simulink model "Regenerative_Brakes_PMSM"  (R2024a)
settings: Solver=ode45  StartTime=0.0  StopTime=2.5  RelTol=1e-3  EnableMultiTasking=on
undefined symbols (not defined in the file): Ion, Lithium, sigbuilder_block
libraries: spsBatteryLib x1, AC7DriveInternalModels x1, spsPermanentMagnetSynchronousMachineLib x1, spsSeriesRLCBranchLib x1, spsThreePhaseFaultLib x1, spsUniversalBridgeLib x1, spspowerguiLib x1
settings Model: Creator=noname  LastModifiedBy=hirah
settings SolverCC: AlgebraicLoopSolver=TrustRegion
settings DataIOCC: LimitDataPoints=on  SaveFormat=Array  ReturnWorkspaceOutputs=off
settings OptimizationCC: LifeSpan=inf
settings DebuggingCC: UnderspecifiedInitializationDetection=Classic  MergeDetectMultiDrivingBlocksExec=none  SolverPrmCheckMsg=warning  UnconnectedInputMsg=warning  UnconnectedOutputMsg=warning  UnconnectedLineMsg=warning  StateNameClashWarn=warning  SFUnexpectedBacktrackingDiag=warning  SFNoUnconditionalDefaultTransitionDiag=warning  SFExecutionAtInitializationDiag=none  ArithmeticOperatorsInVariantConditions=warning
settings HardwareCC: ProdBitPerPointer=32  ProdBitPerSizeT=32  ProdBitPerPtrDiffT=32  ProdLargestAtomicFloat=None  ProdIntDivRoundTo=Undefined  ProdEndianess=Unspecified  ProdWordSize=32  ProdHWDeviceType=32-bit Generic
settings ModelReferenceCC: EnableRefExpFcnMdlSchedulingChecks=on  PropagateSignalLabelsOutOfModel=off
settings SFSimCC: SimUseLocalCustomCode=off  CustomCodeUndefinedFunction=UseInterfaceOnly
settings RTWCC: RTWUseLocalCustomCode=off  GPUComputeCapability=3.5  DLArmComputeVersion=19.05
settings CodeAppCC: StateflowObjectComments=on
settings GRTTargetCC: TargetLangStandard=C89/C90 (ANSI)
settings ConfigComp: CovMetricSettings=dw  CovSaveCumulativeToWorkspaceVar=on  CovSaveSingleToWorkspaceVar=on  CovExternalEMLEnable=off
settings SimscapeCC: SimscapeNormalizeSystem=off

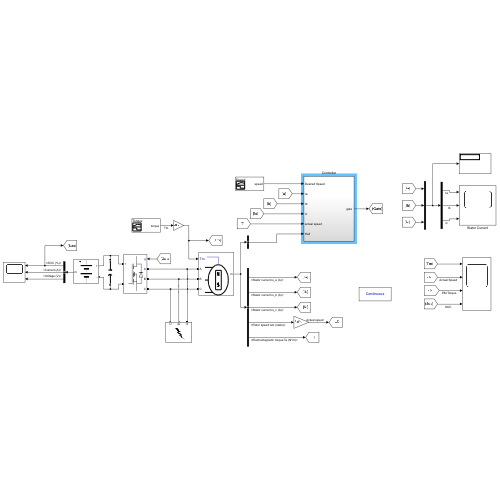
[thumbnail: Simulink's stored preview of the top-level diagram]
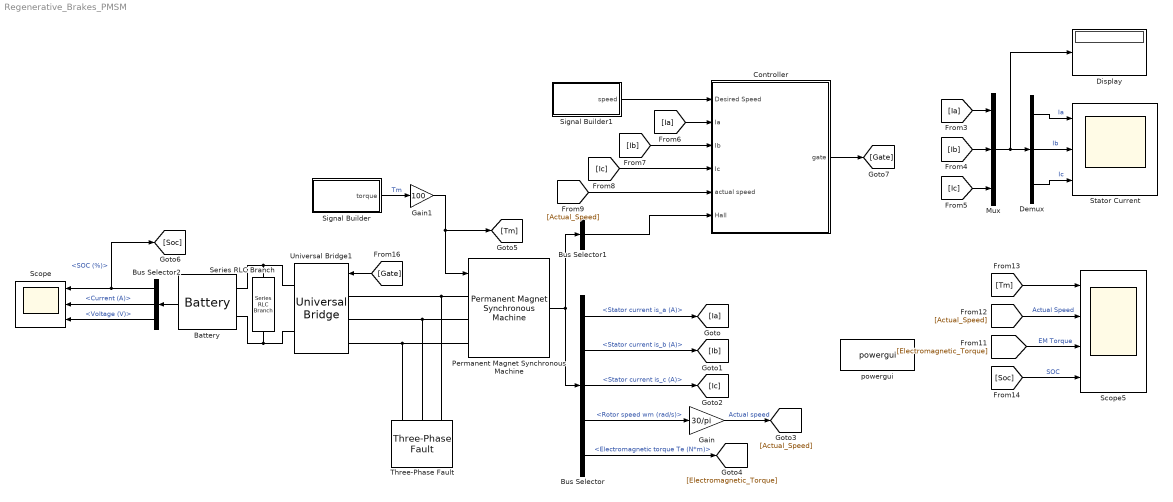
== system Regenerative_Brakes_PMSM ==
  Battery : spsBatteryLib/Battery  BatType=Lithium-Ion  ShowTempParam=off  ThermalPreset=no  ShowAgeParam=off  NomV=300  NomQ=100  SOC=80  Batt_Tr=30  PresetModel=off  MaxQ=84  MinV=215  FullV=330  Dis_rate=27.82608  R=0.006  Normal_OP=57.87524  expZone=[310 3.144344]  current=[1.5 3]  Units=Ampere-hour  Tci=20  NomT=20  T2=-30  MaxQ2=4.8  FullV2=7.1  Normal_OP2=5.655  expZone2="[6.58           1]"  Rca=0.6  ti=2000  Dp=0  Neq0=0  Tsim=1e6  Ta1=25  Qeol=5.4*0.9  Reol=0.013333*1.2  Char_age=[2.3478, 3]  Dis_age=[2.3478, 10]  N1=1500  N2=10500  N3=1000  N4=1400  Ta2=45  N5=950
  Bus Selector : BusSelector  OutputSignals=Stator current is_a (A),Stator current is_b (A),Stator current is_c (A),Rotor speed wm (rad/s),Electromagnetic torque Te (N*m)
  Bus Selector1 : BusSelector  OutputSignals=Hall effect signal h_a,Hall effect signal h_b,Hall effect signal h_c  OutputAsBus=on
  Bus Selector2 : BusSelector  OutputSignals=SOC (%),Current (A),Voltage (V)
  Controller : Subsystem
  Demux : Demux  Outputs=3
  Display : Display
  Gain : Gain  Gain=30/pi
  Gain1 : Gain  Gain=100
  Mux : Mux  Inputs=3
  Permanent Magnet Synchronous Machine : spsPermanentMagnetSynchronousMachineLib/Permanent Magnet Synchronous Machine  NbPhases=3  FluxDistribution=Sinusoidal  RotorType=Round  MechanicalLoad=Torque Tm  PresetModel="07:  20 Nm 300 Vdc 2200 RPM - 33.9 Nm"  ShowDetailedParameters=on  MeasurementBus=off  Resistance=0.129  Inductance=0.0144e-3  dqInductances=[8.5e-3,8.5e-3]  La=0.00153  MachineConstant=Flux linkage established by magnets (V.s)  Flux=0.1821  VoltageCst=132.1171  TorqueCst=1.0926  Flat=120  Mechanical=[0.003334 0.000425 4 0]  PolePairs=4  InitialConditions=[0,0, 0,0]  InitialConditions5ph=[0 0 0 0 0 0]  RefAngle=90 degrees behind phase A axis (modified Park)  IterativeDiscreteModel=Trapezoidal non iterative  TsBlock=-1  TsPowergui=0
  Scope : Scope  NumInputPorts=3
  Scope5 : Scope  NumInputPorts=4
  Series RLC Branch : spsSeriesRLCBranchLib/Series RLC Branch  LConnTagsString=__new0  RConnTagsString=__new0  BranchType=C  Resistance=1  Inductance=1e-3  SetiL0=off  InitialCurrent=0  Capacitance=75e-3  Setx0=off  InitialVoltage=0  Measurements=None
  Signal Builder : Subsystem  Tag=STV Subsys  LoadFcn=sigbuilder_block('load');  StartFcn=sigbuilder_block('start');  StopFcn=sigbuilder_block('stop');  ClipboardFcn=sigbuilder_block('clipboard');  mask(Sigbuilder block){tuvar=[0:10]}
      mask help: Simulink:masks:SigbuilderBlock_MD
      mask init:
      | if ~strcmp(get_param(bdroot(gcbh),'SimulationStatus'),'stopped') tuvar = sigbuilder_block('maskInit'); end
      settings: CopyFcn=sigbuilder_block('copy');  DeleteFcn=sigbuilder_block('delete');  ModelCloseFcn=sigbuilder_block('modelClose');  PreSaveFcn=sigbuilder_block('preSave');  PauseFcn=sigbuilder_block('pause');  ContinueFcn=sigbuilder_block('continue');  NameChangeFcn=sigbuilder_block('namechange');  OpenFcn=sigbuilder_block('open',[437.25 183.75 550.5 395.25 ]);  CloseFcn=sigbuilder_block('close');
      mask Display: plot(0, 0, 100, 100,[2, 2, 32, 32, 2], [68, 8, 8, 68, 68],[32, 2], [38, 38], [32, 19, 2],[53, 60, 44], [32, 17, 17, 2],[16, 16, 31, 31]);txt = getActiveGroup(gcbh);text(2, 100, txt,'verticalAlignment', 'top');
  Signal Builder1 : Subsystem  Tag=STV Subsys  LoadFcn=sigbuilder_block('load');  StartFcn=sigbuilder_block('start');  StopFcn=sigbuilder_block('stop');  ClipboardFcn=sigbuilder_block('clipboard');  mask(Sigbuilder block){tuvar=[0:10]}
      mask help: Simulink:masks:SigbuilderBlock_MD
      mask init:
      | if ~strcmp(get_param(bdroot(gcbh),'SimulationStatus'),'stopped') tuvar = sigbuilder_block('maskInit'); end
      settings: CopyFcn=sigbuilder_block('copy');  DeleteFcn=sigbuilder_block('delete');  ModelCloseFcn=sigbuilder_block('modelClose');  PreSaveFcn=sigbuilder_block('preSave');  PauseFcn=sigbuilder_block('pause');  ContinueFcn=sigbuilder_block('continue');  NameChangeFcn=sigbuilder_block('namechange');  OpenFcn=sigbuilder_block('open',[6.75 6.75 1138.5 568.5 ]);  CloseFcn=sigbuilder_block('close');
      mask Display: plot(0, 0, 100, 100,[2, 2, 32, 32, 2], [68, 8, 8, 68, 68],[32, 2], [38, 38], [32, 19, 2],[53, 60, 44], [32, 17, 17, 2],[16, 16, 31, 31]);txt = getActiveGroup(gcbh);text(2, 100, txt,'verticalAlignment', 'top');
  Stator Current : Scope  NumInputPorts=3
  Three-Phase Fault : spsThreePhaseFaultLib/Three-Phase Fault  InitialStates=0  FaultA=on  FaultB=on  FaultC=on  GroundFault=on  SwitchTimes="[1/60  5/60]"  External=off  SwitchStatus=NaN  FaultResistance=0.001  GroundResistance=0.01  SnubberResistance=1e6  SnubberCapacitance=inf  Measurements=None
  Universal Bridge1 : spsUniversalBridgeLib/Universal Bridge  Arms=3  SnubberResistance=1e5  SnubberCapacitance=inf  Device=MOSFET / Diodes  Ron=1e-3  Lon=0  ForwardVoltages="[  0  0  ]"  ForwardVoltage=0  GTOparameters=[ 10e-6 , 20e-6 ]  IGBTparameters=[ 1e-6 , 2e-6 ]  Measurements=None  Measurements_2=None  converterType=Rectifier
  powergui : spspowerguiLib/powergui  Priority=2  SimulationMode=Continuous  SampleTime=10e-6  frequency=60  Iterations=50  frequencyindice=0  Pbase=100e6  ErrMax=1e-4  UnitsV=kV  UnitsW=MW  buscounter=0  FunctionMessages=off  echomessages=off  EnableUseOfTLC=off  CurrentSourceSwitches=off  DisableSnubberDevices=off  DisableRonSwitches=off  DisableVfSwitches=off  DisplayEquations=off  AutomaticDiscreteSolvers=off  SolverType=Tustin  Interpol=off  ExternalGateDelay=off  methode=off  Ts=0  x0status=blocks  SPID=off  SwTol=0  HookPort=off  NonlinearTolerance=1e-4  nMaxIteration=100  ContinueOnMaxIteration=off  RestoreLinks=warning  ResistiveCurrentMeasurement=off  Frange=[0:2:500]  Ylog=off  Xlog=on  ShowGrid=off  save=off  variable=ZData  structure=N  ZoomFFT=off  StartTime=0.0  cycles=1  DisplayStyle=1  fundamental=60  FreqAxis=off  MaxFrequency=1000  frequencyindicesteady=1  RmsSteady=1  display=off
  wires:
  Permanent Magnet Synchronous Machine/1 -> Bus Selector/1, Bus Selector1/1
  Bus Selector/1 -> [Ia]  "<Stator current is_a (A)>"
  Bus Selector/2 -> [Ib]  "<Stator current is_b (A)>"
  Bus Selector/3 -> [Ic]  "<Stator current is_c (A)>"
  Bus Selector/4 -> Gain/1  "<Rotor speed wm (rad/s)>"
  Bus Selector1/1 -> Controller/6("Hall ")
  Gain/1 -> [Actual_Speed]  "Actual speed"
  Controller/1("gate ") -> [Gate]
  Battery/1 -> Bus Selector2/1
  Bus Selector2/1 -> Scope/1, [Soc]  "<SOC (%)>"
  Bus Selector2/2 -> Scope/2  "<Current (A)>"
  Bus Selector2/3 -> Scope/3  "<Voltage (V)>"
  Mux/1 -> Display/1, Demux/1
  Signal Builder/1(torque) -> Gain1/1  "Tm"
  Bus Selector/5 -> [Electromagnetic_Torque]  "<Electromagnetic torque Te (N*m)>"
  [Ia] -> Mux/1
  [Ib] -> Mux/2
  [Ic] -> Mux/3
  [Ia] -> Controller/2(Ia)
  [Ib] -> Controller/3(Ib)
  [Ic] -> Controller/4(Ic)
  [Actual_Speed] -> Controller/5(actual speed)
  [Actual_Speed] -> Scope5/2  "Actual Speed"
  [Tm] -> Scope5/1
  [Soc] -> Scope5/4  "SOC"
  [Gate] -> Universal Bridge1/1
  Signal Builder1/1(speed) -> Controller/1(Desired Speed)
  Demux/1 -> Stator Current/1  "Ia"
  Demux/2 -> Stator Current/2  "Ib"
  Demux/3 -> Stator Current/3  "Ic"
  [Electromagnetic_Torque] -> Scope5/3  "EM Torque"
  Gain1/1 -> Permanent Magnet Synchronous Machine/1, [Tm]
  connections:
  Universal Bridge1/LConn1 -- Three-Phase Fault/LConn1 -- Permanent Magnet Synchronous Machine/LConn1
  Permanent Magnet Synchronous Machine/LConn2 -- Universal Bridge1/LConn2 -- Three-Phase Fault/LConn2
  Universal Bridge1/LConn3 -- Three-Phase Fault/LConn3 -- Permanent Magnet Synchronous Machine/LConn3
  Series RLC Branch/LConn1 -- Universal Bridge1/RConn1 -- Battery/LConn1
  Series RLC Branch/RConn1 -- Battery/LConn2 -- Universal Bridge1/RConn2

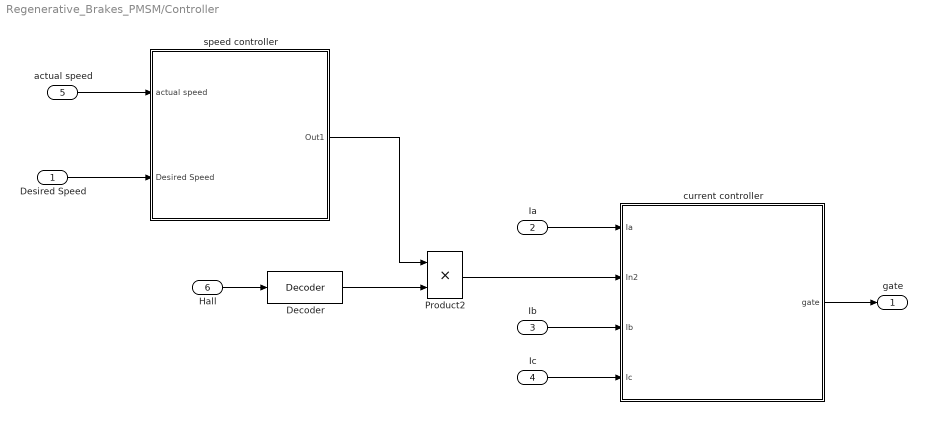
== system Regenerative_Brakes_PMSM/Controller ==
  Desired Speed : Inport
  Ia : Inport  Port=2
  Ib : Inport  Port=3
  Ic : Inport  Port=4
  actual speed : Inport  Port=5
  "Hall " : Inport  Port=6
  Decoder : AC7DriveInternalModels/Current Controller/Decoder  SystemSampleTime=-1  VariantActivationTime=update diagram  AllowFlexibleInterface=on  Latency=0  AutoFrameSizeCalculation=off
  Product2 : Product  SaturateOnIntegerOverflow=on  OutDataTypeStr=Inherit: Same as first input
  current controller : Subsystem
  speed controller : Subsystem
  "gate " : Outport  VectorParamsAs1DForOutWhenUnconnected=off
  wires:
  "Hall "/1 -> Decoder/1
  Decoder/1 -> Product2/2
  current controller/1("gate ") -> "gate "/1
  Ic/1 -> current controller/4(Ic)
  Ib/1 -> current controller/3(Ib)
  Ia/1 -> current controller/1(Ia)
  Product2/1 -> current controller/2(In2)
  actual speed/1 -> speed controller/1(actual speed)
  speed controller/1(Out1) -> Product2/1
  Desired Speed/1 -> speed controller/2(Desired Speed)

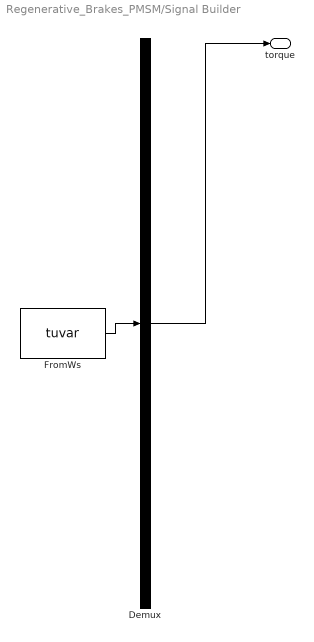
== system Regenerative_Brakes_PMSM/Signal Builder ==
  Demux : Demux  Tag=STV Demux  Outputs=1
      settings: DisplayOption=none
  FromWs : FromWorkspace  Tag=STV FromWs  VariableName=tuvar
      SigBuilderData=|
      | common.afterFinalStr = 'Extrapolate'
      | common.sampleTime = 0
      | dataSet.timeRange = [0 2.5]
      | dataSet.name = 'Torque'
      | sbobj.Name = 'Signal Builder'
      | sbobj.Groups.Name = 'Torque'
      | sbobj.Groups.Signals.Name = 'torque'
      | sbobj.Groups.Signals.XData = [0 0.05 0.05 0.5 0.5 0.75 0.75 1.25 1.25 1.65 1.65 2.05 2.05 2.35 2.35 2.5]
      | sbobj.Groups.Signals.YData = [0 0 5 5 -1 -1 -3 -3 1.5 1.5 5 5 4 4 -1 -1]
      | sbobj.Groups.TimeRange = [0 2.5]
  torque : Outport  VectorParamsAs1DForOutWhenUnconnected=off
  wires:
  Demux/1 -> torque/1
  FromWs/1 -> Demux/1

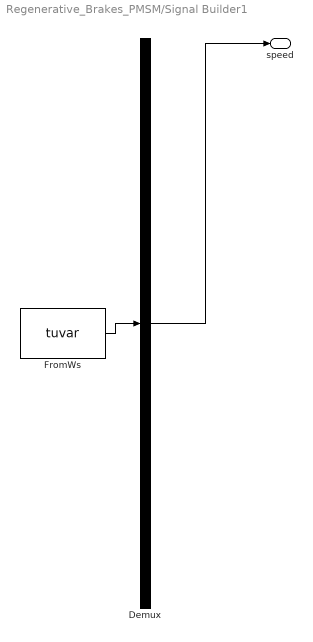
== system Regenerative_Brakes_PMSM/Signal Builder1 ==
  Demux : Demux  Tag=STV Demux  Outputs=1
      settings: DisplayOption=none
  FromWs : FromWorkspace  Tag=STV FromWs  VariableName=tuvar
      SigBuilderData=|
      | common.afterFinalStr = 'Extrapolate'
      | common.sampleTime = 0
      | dataSet.timeRange = [0 2.5]
      | dataSet.name = 'Speed'
      | sbobj.Name = 'Signal Builder'
      | sbobj.Groups.Name = 'Speed'
      | sbobj.Groups.Signals.Name = 'speed'
      | sbobj.Groups.Signals.XData = [0 0.05 0.5 0.75 1 1.5 2 2.35 2.5]
      | sbobj.Groups.Signals.YData = [0 0 2500 2500 1000 1000 2000 2000 1000]
      | sbobj.Groups.TimeRange = [0 2.5]
  speed : Outport  VectorParamsAs1DForOutWhenUnconnected=off
  wires:
  Demux/1 -> speed/1
  FromWs/1 -> Demux/1

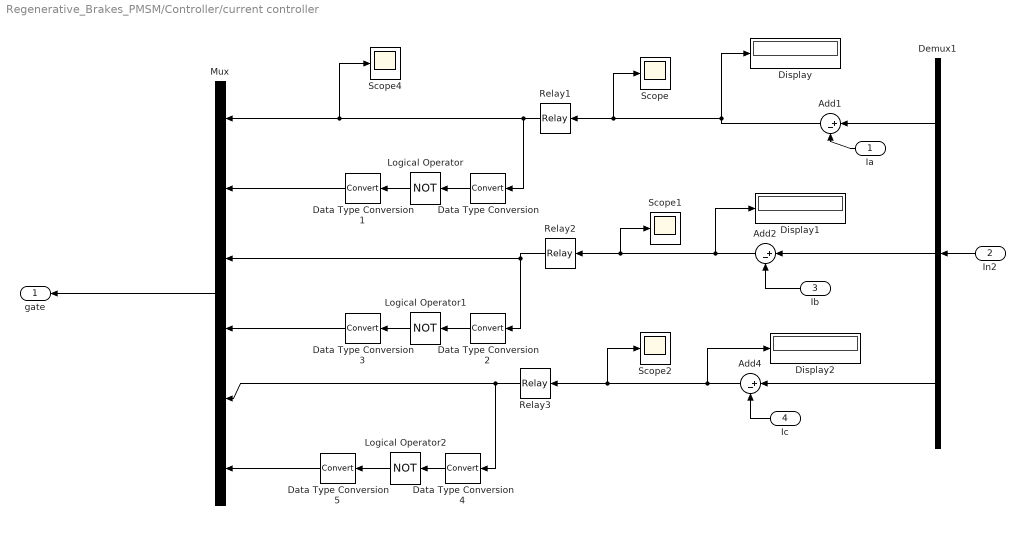
== system Regenerative_Brakes_PMSM/Controller/current controller ==
  Ia : Inport
  In2 : Inport  Port=2
  Ib : Inport  Port=3
  Ic : Inport  Port=4
  Add1 : Sum  Inputs=|+-
  Add2 : Sum  Inputs=|+-
  Add4 : Sum  Inputs=|+-
  Data Type Conversion{,1..5} (6 alike) : DataTypeConversion
  Demux1 : Demux  Outputs=3
      settings: DisplayOption=none
  Display : Display
  Display1 : Display
  Display2 : Display
  Logical Operator : Logic  Operator=NOT  AllPortsSameDT=off  OutDataTypeStr=boolean
  Logical Operator1 : Logic  Operator=NOT  AllPortsSameDT=off  OutDataTypeStr=boolean
  Logical Operator2 : Logic  Operator=NOT  AllPortsSameDT=off  OutDataTypeStr=boolean
  Mux : Mux  Inputs=6
  Relay1 : Relay  OnSwitchValue=5  OffSwitchValue=-5
  Relay2 : Relay  OnSwitchValue=5  OffSwitchValue=-5
  Relay3 : Relay  OnSwitchValue=5  OffSwitchValue=-5
  Scope{,1..2,4} (4 alike) : Scope
  "gate " : Outport  VectorParamsAs1DForOutWhenUnconnected=off
  wires:
  Relay1/1 -> Scope4/1, Mux/1, Data Type Conversion/1
  Relay2/1 -> Mux/3, Data Type Conversion2/1
  Relay3/1 -> Mux/5, Data Type Conversion4/1
  Ib/1 -> Add2/2
  Mux/1 -> "gate "/1
  Ic/1 -> Add4/2
  Add4/1 -> Display2/1, Scope2/1, Relay3/1
  Add2/1 -> Relay2/1, Scope1/1, Display1/1
  Add1/1 -> Display/1, Scope/1, Relay1/1
  Data Type Conversion/1 -> Logical Operator/1
  Logical Operator/1 -> Data Type Conversion1/1
  Data Type Conversion1/1 -> Mux/2
  Logical Operator1/1 -> Data Type Conversion3/1
  Data Type Conversion3/1 -> Mux/4
  Data Type Conversion2/1 -> Logical Operator1/1
  Data Type Conversion5/1 -> Mux/6
  Logical Operator2/1 -> Data Type Conversion5/1
  Data Type Conversion4/1 -> Logical Operator2/1
  Demux1/2 -> Add2/1
  Demux1/3 -> Add4/1
  In2/1 -> Demux1/1
  Ia/1 -> Add1/2
  Demux1/1 -> Add1/1

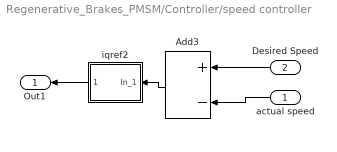
== system Regenerative_Brakes_PMSM/Controller/speed controller ==
  actual speed : Inport
  Desired Speed : Inport  Port=2
  Add3 : Sum  Inputs=+-
  iqref2 : Subsystem  mask(PI Controller){I=2.8, P=5, sat=[-inf, inf]}
      mask prompts: I "Integral"; P "Proportional:"; sat "Minimum and maximum outputs:"
      mask init:
      | min=sat(1);max=sat(2);
      mask Display: disp('PI')
  Out1 : Outport  VectorParamsAs1DForOutWhenUnconnected=off
  wires:
  actual speed/1 -> Add3/2
  Desired Speed/1 -> Add3/1
  Add3/1 -> iqref2/1(In_1)
  iqref2/1(Out_1) -> Out1/1

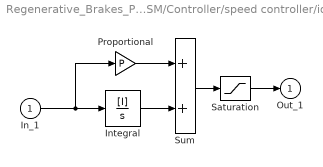
== system Regenerative_Brakes_PMSM/Controller/speed controller/iqref2 ==
  In_1 : Inport
  Integral : TransferFcn  Numerator=[I]  Denominator=[1 0]
  Proportional : Gain  Gain=P  SaturateOnIntegerOverflow=on  OutDataTypeStr=Inherit: Same as input  ParamDataTypeStr=Inherit: Same as input
  Saturation : Saturate  UpperLimit=max  LowerLimit=min
  Sum : Sum  InputSameDT=on  SaturateOnIntegerOverflow=on  OutDataTypeStr=Inherit: Same as first input
  Out_1 : Outport  InitialOutput=0  VectorParamsAs1DForOutWhenUnconnected=off
  wires:
  Integral/1 -> Sum/2
  In_1/1 -> Integral/1, Proportional/1
  Proportional/1 -> Sum/1
  Sum/1 -> Saturation/1
  Saturation/1 -> Out_1/1
